simulink model "simulation_4_constant_capacity"  (R2026a)
settings: Solver=VariableStepAuto  StopTime=12000
undefined symbols (not defined in the file): battery_builder_rtmsupport, gcbh
libraries: fl_lib x36, nesl_utility x18, BatteryCurrentManagement x6, Batteries_lib x6, BatteryEstimators x6
(part 2 of 2)

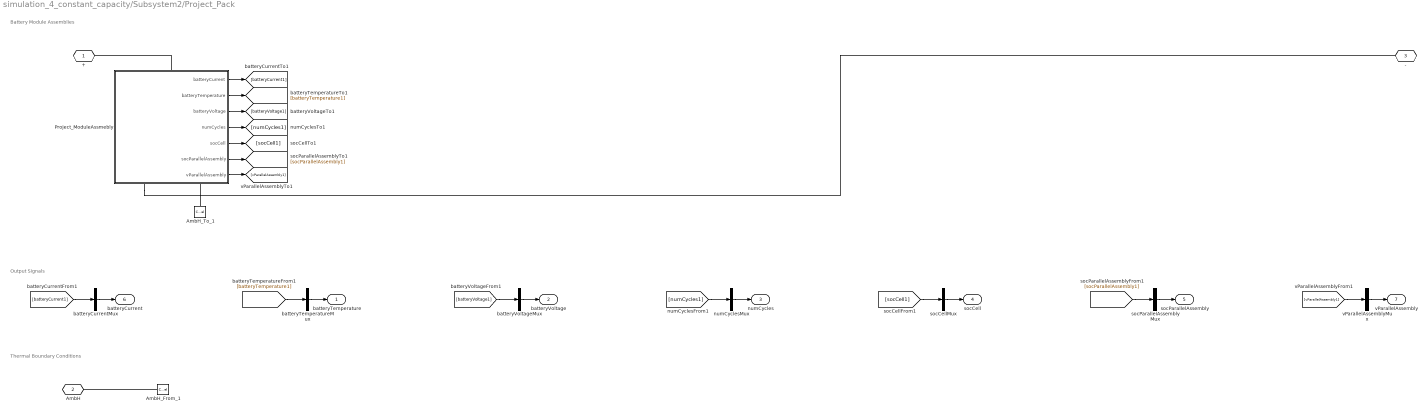
== system simulation_4_constant_capacity/Subsystem2/Project_Pack ==
  note: Thermal Boundary Conditions
  note: Output Signals
  note: Battery Module Assemblies
  AmbH_From_1 : ConnectionLabel  Label=ambH_1
  AmbH_To_1 : ConnectionLabel  Label=ambH_1
  Project_ModuleAssmebly : Subsystem  LoadFcn=battery_builder_rtmsupport('loadfcn',gcbh);
      settings: CopyFcn=battery_builder_rtmsupport('copyfcn',gcbh);  PreCopyFcn=battery_builder_rtmsupport('precopyfcn',gcbh);  PreDeleteFcn=battery_builder_rtmsupport('predeletefcn',gcbh);  PortSchema="{\"entries\":[{\"content\":{\"sides\":[{\"content\":{\"connectorIds\":[\"LConn1\"]},\"type\":\"ConnectorPlacement.EquallySpacedRectSide\",\"uuid\":\"76c6f046-db8e-4015-a922-00ba973faf16\"},{\"content\":{\"connectorIds\":[\"RConn1\",\"RConn2\"],\"side\":\"RIGHT\"},\"type\":\"ConnectorPlacement.EquallySpacedRectSide\",\"uuid\":\"59fdee5c-a6f4-4b44-aa6e-82d2d9418fce\"},{\"content\":{\"side\":\"TOP\"},\"type\":\"ConnectorPlacement.EquallySpacedRectSide\",\"uuid\":\"84b83595-cc1f-46da-a2b0-c16634a6daab\"},{\"content\":{\"connectorIds\":[\"Out1\",\"Out2\",\"Out3\",\"Out4\",\"Out5\",\"Out6\",\"Out7\"],\"side\":\"BOTTOM\"},\"type\":\"ConnectorPlacement.EquallySpacedRectSide\",\"uuid\":\"391f6102-8f79-4306-a331-0bb83eeeb4a2\"}]},\"type\":\"ConnectorPlacement.EquallySpacedConnector\",\"uuid\":\"e6fb231a-8daf-4bfc-bdc1-9175fa7a2dfd\"}],\"packageUris\":[\"http://schema.mathworks.com/mf0/Connector/R2020b\"],\"version\":\"1.0\"}"
      mask Display: image('$imagefile')
  batteryCurrentMux : Mux  Inputs=1
  batteryTemperatureMux : Mux  Inputs=1
  batteryVoltageMux : Mux  Inputs=1
  numCyclesMux : Mux  Inputs=1
  socCellMux : Mux  Inputs=1
  socParallelAssemblyMux : Mux  Inputs=1
  vParallelAssemblyMux : Mux  Inputs=1
  + : PMIOPort  Side=Left
  AmbH : PMIOPort  Port=2  Side=Right  ConnectionType=Connection: foundation.thermal.thermal
  - : PMIOPort  Port=3  Side=Right
  batteryTemperature : Outport
  batteryVoltage : Outport  Port=2
  numCycles : Outport  Port=3
  socCell : Outport  Port=4
  socParallelAssembly : Outport  Port=5
  batteryCurrent : Outport  Port=6
  vParallelAssembly : Outport  Port=7
  wires:
  [vParallelAssembly1] -> vParallelAssemblyMux/1
  vParallelAssemblyMux/1 -> vParallelAssembly/1
  Project_ModuleAssmebly/7(vParallelAssembly) -> [vParallelAssembly1]
  [socParallelAssembly1] -> socParallelAssemblyMux/1
  socParallelAssemblyMux/1 -> socParallelAssembly/1
  Project_ModuleAssmebly/6(socParallelAssembly) -> [socParallelAssembly1]
  [socCell1] -> socCellMux/1
  socCellMux/1 -> socCell/1
  Project_ModuleAssmebly/5(socCell) -> [socCell1]
  [numCycles1] -> numCyclesMux/1
  numCyclesMux/1 -> numCycles/1
  Project_ModuleAssmebly/4(numCycles) -> [numCycles1]
  [batteryVoltage1] -> batteryVoltageMux/1
  batteryVoltageMux/1 -> batteryVoltage/1
  Project_ModuleAssmebly/3(batteryVoltage) -> [batteryVoltage1]
  [batteryTemperature1] -> batteryTemperatureMux/1
  batteryTemperatureMux/1 -> batteryTemperature/1
  Project_ModuleAssmebly/2(batteryTemperature) -> [batteryTemperature1]
  [batteryCurrent1] -> batteryCurrentMux/1
  batteryCurrentMux/1 -> batteryCurrent/1
  Project_ModuleAssmebly/1(batteryCurrent) -> [batteryCurrent1]
  connections:
  AmbH_From_1/LConn1 -- AmbH/RConn1
  AmbH_To_1/LConn1 -- Project_ModuleAssmebly/RConn2
  Project_ModuleAssmebly/RConn1 -- -/RConn1
  Project_ModuleAssmebly/LConn1 -- +/RConn1

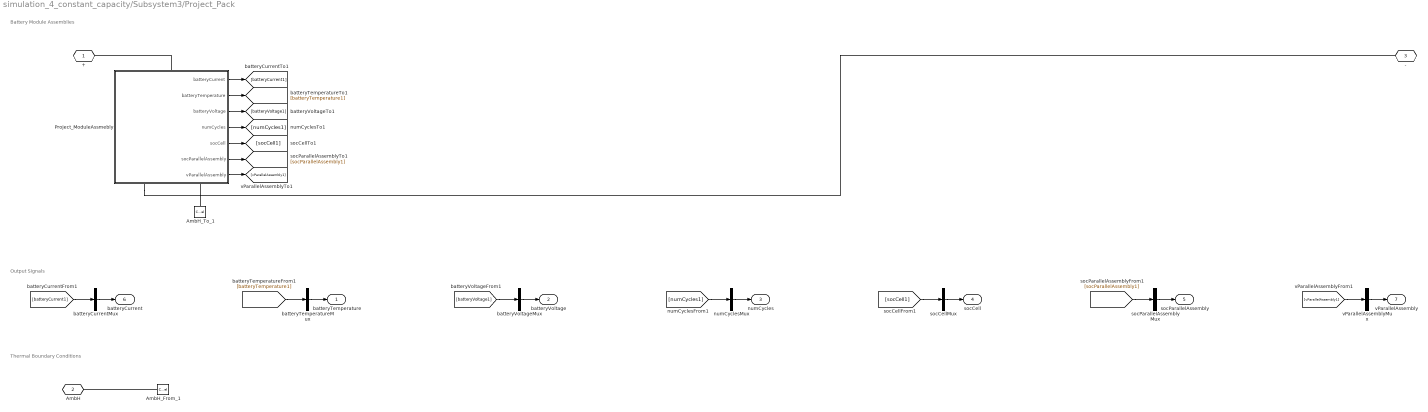
== system simulation_4_constant_capacity/Subsystem3/Project_Pack ==
  note: Thermal Boundary Conditions
  note: Output Signals
  note: Battery Module Assemblies
  AmbH_From_1 : ConnectionLabel  Label=ambH_1
  AmbH_To_1 : ConnectionLabel  Label=ambH_1
  Project_ModuleAssmebly : Subsystem  LoadFcn=battery_builder_rtmsupport('loadfcn',gcbh);
      settings: CopyFcn=battery_builder_rtmsupport('copyfcn',gcbh);  PreCopyFcn=battery_builder_rtmsupport('precopyfcn',gcbh);  PreDeleteFcn=battery_builder_rtmsupport('predeletefcn',gcbh);  PortSchema="{\"entries\":[{\"content\":{\"sides\":[{\"content\":{\"connectorIds\":[\"LConn1\"]},\"type\":\"ConnectorPlacement.EquallySpacedRectSide\",\"uuid\":\"76c6f046-db8e-4015-a922-00ba973faf16\"},{\"content\":{\"connectorIds\":[\"RConn1\",\"RConn2\"],\"side\":\"RIGHT\"},\"type\":\"ConnectorPlacement.EquallySpacedRectSide\",\"uuid\":\"59fdee5c-a6f4-4b44-aa6e-82d2d9418fce\"},{\"content\":{\"side\":\"TOP\"},\"type\":\"ConnectorPlacement.EquallySpacedRectSide\",\"uuid\":\"84b83595-cc1f-46da-a2b0-c16634a6daab\"},{\"content\":{\"connectorIds\":[\"Out1\",\"Out2\",\"Out3\",\"Out4\",\"Out5\",\"Out6\",\"Out7\"],\"side\":\"BOTTOM\"},\"type\":\"ConnectorPlacement.EquallySpacedRectSide\",\"uuid\":\"391f6102-8f79-4306-a331-0bb83eeeb4a2\"}]},\"type\":\"ConnectorPlacement.EquallySpacedConnector\",\"uuid\":\"e6fb231a-8daf-4bfc-bdc1-9175fa7a2dfd\"}],\"packageUris\":[\"http://schema.mathworks.com/mf0/Connector/R2020b\"],\"version\":\"1.0\"}"
      mask Display: image('$imagefile')
  batteryCurrentMux : Mux  Inputs=1
  batteryTemperatureMux : Mux  Inputs=1
  batteryVoltageMux : Mux  Inputs=1
  numCyclesMux : Mux  Inputs=1
  socCellMux : Mux  Inputs=1
  socParallelAssemblyMux : Mux  Inputs=1
  vParallelAssemblyMux : Mux  Inputs=1
  + : PMIOPort  Side=Left
  AmbH : PMIOPort  Port=2  Side=Right  ConnectionType=Connection: foundation.thermal.thermal
  - : PMIOPort  Port=3  Side=Right
  batteryTemperature : Outport
  batteryVoltage : Outport  Port=2
  numCycles : Outport  Port=3
  socCell : Outport  Port=4
  socParallelAssembly : Outport  Port=5
  batteryCurrent : Outport  Port=6
  vParallelAssembly : Outport  Port=7
  wires:
  [vParallelAssembly1] -> vParallelAssemblyMux/1
  vParallelAssemblyMux/1 -> vParallelAssembly/1
  Project_ModuleAssmebly/7(vParallelAssembly) -> [vParallelAssembly1]
  [socParallelAssembly1] -> socParallelAssemblyMux/1
  socParallelAssemblyMux/1 -> socParallelAssembly/1
  Project_ModuleAssmebly/6(socParallelAssembly) -> [socParallelAssembly1]
  [socCell1] -> socCellMux/1
  socCellMux/1 -> socCell/1
  Project_ModuleAssmebly/5(socCell) -> [socCell1]
  [numCycles1] -> numCyclesMux/1
  numCyclesMux/1 -> numCycles/1
  Project_ModuleAssmebly/4(numCycles) -> [numCycles1]
  [batteryVoltage1] -> batteryVoltageMux/1
  batteryVoltageMux/1 -> batteryVoltage/1
  Project_ModuleAssmebly/3(batteryVoltage) -> [batteryVoltage1]
  [batteryTemperature1] -> batteryTemperatureMux/1
  batteryTemperatureMux/1 -> batteryTemperature/1
  Project_ModuleAssmebly/2(batteryTemperature) -> [batteryTemperature1]
  [batteryCurrent1] -> batteryCurrentMux/1
  batteryCurrentMux/1 -> batteryCurrent/1
  Project_ModuleAssmebly/1(batteryCurrent) -> [batteryCurrent1]
  connections:
  AmbH_From_1/LConn1 -- AmbH/RConn1
  AmbH_To_1/LConn1 -- Project_ModuleAssmebly/RConn2
  Project_ModuleAssmebly/RConn1 -- -/RConn1
  Project_ModuleAssmebly/LConn1 -- +/RConn1

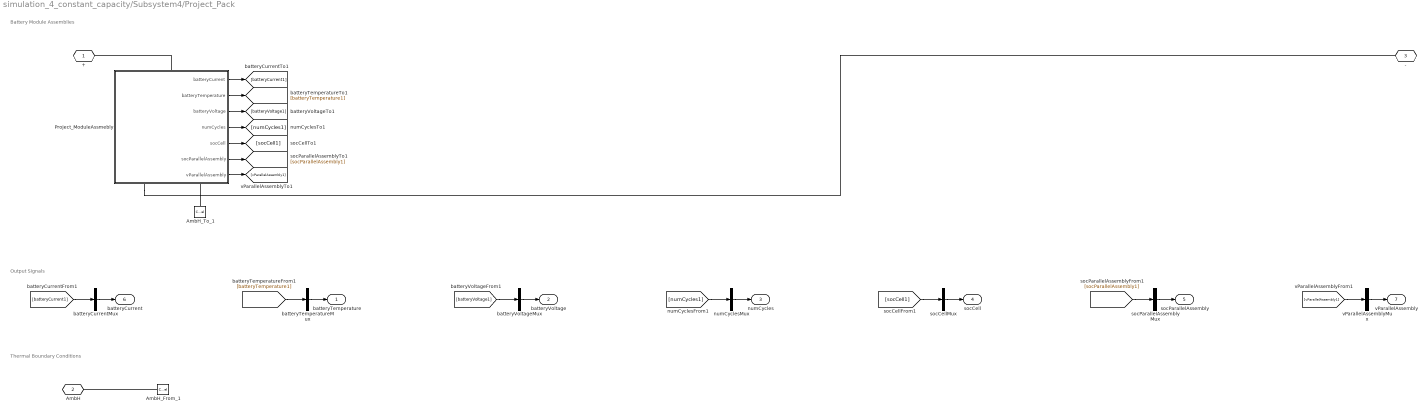
== system simulation_4_constant_capacity/Subsystem4/Project_Pack ==
  note: Thermal Boundary Conditions
  note: Output Signals
  note: Battery Module Assemblies
  AmbH_From_1 : ConnectionLabel  Label=ambH_1
  AmbH_To_1 : ConnectionLabel  Label=ambH_1
  Project_ModuleAssmebly : Subsystem  LoadFcn=battery_builder_rtmsupport('loadfcn',gcbh);
      settings: CopyFcn=battery_builder_rtmsupport('copyfcn',gcbh);  PreCopyFcn=battery_builder_rtmsupport('precopyfcn',gcbh);  PreDeleteFcn=battery_builder_rtmsupport('predeletefcn',gcbh);  PortSchema="{\"entries\":[{\"content\":{\"sides\":[{\"content\":{\"connectorIds\":[\"LConn1\"]},\"type\":\"ConnectorPlacement.EquallySpacedRectSide\",\"uuid\":\"76c6f046-db8e-4015-a922-00ba973faf16\"},{\"content\":{\"connectorIds\":[\"RConn1\",\"RConn2\"],\"side\":\"RIGHT\"},\"type\":\"ConnectorPlacement.EquallySpacedRectSide\",\"uuid\":\"59fdee5c-a6f4-4b44-aa6e-82d2d9418fce\"},{\"content\":{\"side\":\"TOP\"},\"type\":\"ConnectorPlacement.EquallySpacedRectSide\",\"uuid\":\"84b83595-cc1f-46da-a2b0-c16634a6daab\"},{\"content\":{\"connectorIds\":[\"Out1\",\"Out2\",\"Out3\",\"Out4\",\"Out5\",\"Out6\",\"Out7\"],\"side\":\"BOTTOM\"},\"type\":\"ConnectorPlacement.EquallySpacedRectSide\",\"uuid\":\"391f6102-8f79-4306-a331-0bb83eeeb4a2\"}]},\"type\":\"ConnectorPlacement.EquallySpacedConnector\",\"uuid\":\"e6fb231a-8daf-4bfc-bdc1-9175fa7a2dfd\"}],\"packageUris\":[\"http://schema.mathworks.com/mf0/Connector/R2020b\"],\"version\":\"1.0\"}"
      mask Display: image('$imagefile')
  batteryCurrentMux : Mux  Inputs=1
  batteryTemperatureMux : Mux  Inputs=1
  batteryVoltageMux : Mux  Inputs=1
  numCyclesMux : Mux  Inputs=1
  socCellMux : Mux  Inputs=1
  socParallelAssemblyMux : Mux  Inputs=1
  vParallelAssemblyMux : Mux  Inputs=1
  + : PMIOPort  Side=Left
  AmbH : PMIOPort  Port=2  Side=Right  ConnectionType=Connection: foundation.thermal.thermal
  - : PMIOPort  Port=3  Side=Right
  batteryTemperature : Outport
  batteryVoltage : Outport  Port=2
  numCycles : Outport  Port=3
  socCell : Outport  Port=4
  socParallelAssembly : Outport  Port=5
  batteryCurrent : Outport  Port=6
  vParallelAssembly : Outport  Port=7
  wires:
  [vParallelAssembly1] -> vParallelAssemblyMux/1
  vParallelAssemblyMux/1 -> vParallelAssembly/1
  Project_ModuleAssmebly/7(vParallelAssembly) -> [vParallelAssembly1]
  [socParallelAssembly1] -> socParallelAssemblyMux/1
  socParallelAssemblyMux/1 -> socParallelAssembly/1
  Project_ModuleAssmebly/6(socParallelAssembly) -> [socParallelAssembly1]
  [socCell1] -> socCellMux/1
  socCellMux/1 -> socCell/1
  Project_ModuleAssmebly/5(socCell) -> [socCell1]
  [numCycles1] -> numCyclesMux/1
  numCyclesMux/1 -> numCycles/1
  Project_ModuleAssmebly/4(numCycles) -> [numCycles1]
  [batteryVoltage1] -> batteryVoltageMux/1
  batteryVoltageMux/1 -> batteryVoltage/1
  Project_ModuleAssmebly/3(batteryVoltage) -> [batteryVoltage1]
  [batteryTemperature1] -> batteryTemperatureMux/1
  batteryTemperatureMux/1 -> batteryTemperature/1
  Project_ModuleAssmebly/2(batteryTemperature) -> [batteryTemperature1]
  [batteryCurrent1] -> batteryCurrentMux/1
  batteryCurrentMux/1 -> batteryCurrent/1
  Project_ModuleAssmebly/1(batteryCurrent) -> [batteryCurrent1]
  connections:
  AmbH_From_1/LConn1 -- AmbH/RConn1
  AmbH_To_1/LConn1 -- Project_ModuleAssmebly/RConn2
  Project_ModuleAssmebly/RConn1 -- -/RConn1
  Project_ModuleAssmebly/LConn1 -- +/RConn1

== system simulation_4_constant_capacity/Subsystem5/Project_Pack ==
  note: Thermal Boundary Conditions
  note: Output Signals
  note: Battery Module Assemblies
  AmbH_From_1 : ConnectionLabel  Label=ambH_1
  AmbH_To_1 : ConnectionLabel  Label=ambH_1
  Project_ModuleAssmebly : Subsystem  LoadFcn=battery_builder_rtmsupport('loadfcn',gcbh);
      settings: CopyFcn=battery_builder_rtmsupport('copyfcn',gcbh);  PreCopyFcn=battery_builder_rtmsupport('precopyfcn',gcbh);  PreDeleteFcn=battery_builder_rtmsupport('predeletefcn',gcbh);  PortSchema="{\"entries\":[{\"content\":{\"sides\":[{\"content\":{\"connectorIds\":[\"LConn1\"]},\"type\":\"ConnectorPlacement.EquallySpacedRectSide\",\"uuid\":\"76c6f046-db8e-4015-a922-00ba973faf16\"},{\"content\":{\"connectorIds\":[\"RConn1\",\"RConn2\"],\"side\":\"RIGHT\"},\"type\":\"ConnectorPlacement.EquallySpacedRectSide\",\"uuid\":\"59fdee5c-a6f4-4b44-aa6e-82d2d9418fce\"},{\"content\":{\"side\":\"TOP\"},\"type\":\"ConnectorPlacement.EquallySpacedRectSide\",\"uuid\":\"84b83595-cc1f-46da-a2b0-c16634a6daab\"},{\"content\":{\"connectorIds\":[\"Out1\",\"Out2\",\"Out3\",\"Out4\",\"Out5\",\"Out6\",\"Out7\"],\"side\":\"BOTTOM\"},\"type\":\"ConnectorPlacement.EquallySpacedRectSide\",\"uuid\":\"391f6102-8f79-4306-a331-0bb83eeeb4a2\"}]},\"type\":\"ConnectorPlacement.EquallySpacedConnector\",\"uuid\":\"e6fb231a-8daf-4bfc-bdc1-9175fa7a2dfd\"}],\"packageUris\":[\"http://schema.mathworks.com/mf0/Connector/R2020b\"],\"version\":\"1.0\"}"
      mask Display: image('$imagefile')
  batteryCurrentMux : Mux  Inputs=1
  batteryTemperatureMux : Mux  Inputs=1
  batteryVoltageMux : Mux  Inputs=1
  numCyclesMux : Mux  Inputs=1
  socCellMux : Mux  Inputs=1
  socParallelAssemblyMux : Mux  Inputs=1
  vParallelAssemblyMux : Mux  Inputs=1
  + : PMIOPort  Side=Left
  AmbH : PMIOPort  Port=2  Side=Right  ConnectionType=Connection: foundation.thermal.thermal
  - : PMIOPort  Port=3  Side=Right
  batteryTemperature : Outport
  batteryVoltage : Outport  Port=2
  numCycles : Outport  Port=3
  socCell : Outport  Port=4
  socParallelAssembly : Outport  Port=5
  batteryCurrent : Outport  Port=6
  vParallelAssembly : Outport  Port=7
  wires:
  [vParallelAssembly1] -> vParallelAssemblyMux/1
  vParallelAssemblyMux/1 -> vParallelAssembly/1
  Project_ModuleAssmebly/7(vParallelAssembly) -> [vParallelAssembly1]
  [socParallelAssembly1] -> socParallelAssemblyMux/1
  socParallelAssemblyMux/1 -> socParallelAssembly/1
  Project_ModuleAssmebly/6(socParallelAssembly) -> [socParallelAssembly1]
  [socCell1] -> socCellMux/1
  socCellMux/1 -> socCell/1
  Project_ModuleAssmebly/5(socCell) -> [socCell1]
  [numCycles1] -> numCyclesMux/1
  numCyclesMux/1 -> numCycles/1
  Project_ModuleAssmebly/4(numCycles) -> [numCycles1]
  [batteryVoltage1] -> batteryVoltageMux/1
  batteryVoltageMux/1 -> batteryVoltage/1
  Project_ModuleAssmebly/3(batteryVoltage) -> [batteryVoltage1]
  [batteryTemperature1] -> batteryTemperatureMux/1
  batteryTemperatureMux/1 -> batteryTemperature/1
  Project_ModuleAssmebly/2(batteryTemperature) -> [batteryTemperature1]
  [batteryCurrent1] -> batteryCurrentMux/1
  batteryCurrentMux/1 -> batteryCurrent/1
  Project_ModuleAssmebly/1(batteryCurrent) -> [batteryCurrent1]
  connections:
  AmbH_From_1/LConn1 -- AmbH/RConn1
  AmbH_To_1/LConn1 -- Project_ModuleAssmebly/RConn2
  Project_ModuleAssmebly/RConn1 -- -/RConn1
  Project_ModuleAssmebly/LConn1 -- +/RConn1

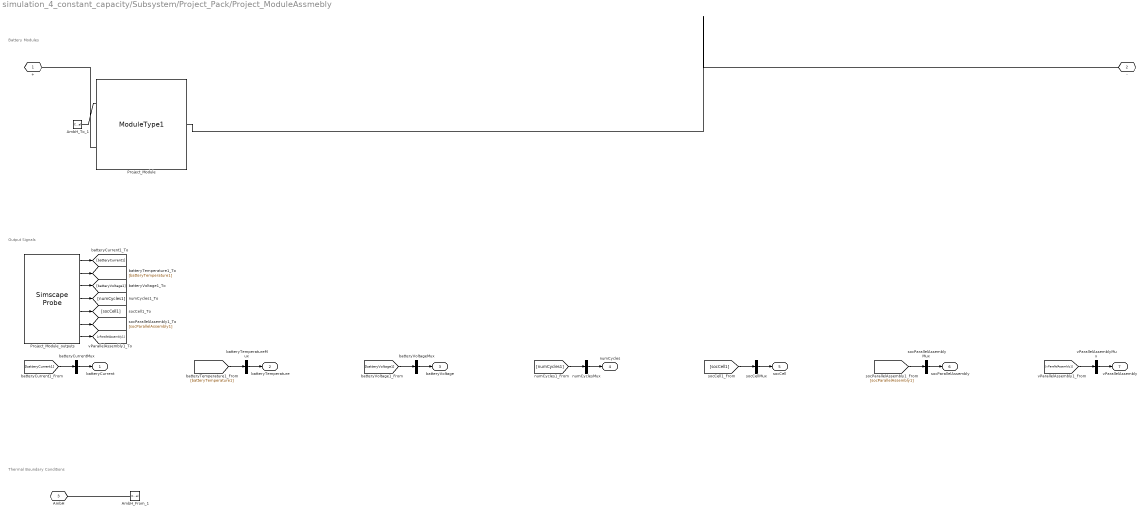
== system simulation_4_constant_capacity/Subsystem/Project_Pack/Project_ModuleAssmebly ==
  note: Battery Modules
  note: Output Signals
  note: Thermal Boundary Conditions
  AmbH_From_1 : ConnectionLabel  Label=ambH_1
  AmbH_To_1 : ConnectionLabel  Label=ambH_1
  Project_Module : Batteries_lib/Modules/ModuleType1  BatteryCapacityCell=2.6 A*hr  ExtrapolationMethodCell=simscape.enum.extrapolation.nearest  SOCBreakpointsCell=[0 0.1 0.2 0.3 0.4 0.5 0.6 0.7 0.8 0.9 1]  TemperatureBreakpointsCell=[253.15 263.15 273.15 296.15 318.15] K  OpenCircuitVoltageThermalCell=|  VoltageRangeCell=[0, inf] V  ResistanceSOCBreakpointsCell=[0, .1, .25, .5, .75, .9, 1]  ResistanceTemperatureBreakpointsCell=[278, 293, 313] K  R0ThermalCell=[.0117, .0085, .009; .011, .0085, .009; .0114, .0087, .0092; .0107, .0082, .0088; .0107, .0083, .0091; .0113, .0085, .0089; .0116, .0085, .0089] Ohm  BatteryThermalMassCell=1840 J/K  AmbientResistance=25 K/W  socCell_specify=off  socCell_priority=High  socCell=0  socCell_nominal_specify=off  socCell_nominal_value=1  socCell_nominal_unit=1  batteryVoltage_specify=off  batteryVoltage_priority=None  batteryVoltage=0 V  batteryVoltage_nominal_specify=off  batteryVoltage_nominal_value=1  batteryVoltage_nominal_unit=V  batteryCurrent_specify=off  batteryCurrent_priority=None  batteryCurrent=0 A  batteryCurrent_nominal_specify=off  batteryCurrent_nominal_value=1  batteryCurrent_nominal_unit=A  numCycles_specify=off  numCycles_priority=High  numCycles=0  numCycles_nominal_specify=off  numCycles_nominal_value=1  numCycles_nominal_unit=1  batteryTemperature_specify=on  batteryTemperature_priority=High  batteryTemperature=258 K  batteryTemperature_nominal_specify=off  batteryTemperature_nominal_value=1  batteryTemperature_nominal_unit=K  vParallelAssembly_specify=off  vParallelAssembly_priority=None  vParallelAssembly=repmat(0, 10, 1) V  vParallelAssembly_nominal_specify=off  vParallelAssembly_nominal_value=1  vParallelAssembly_nominal_unit=V  socParallelAssembly_specify=off  socParallelAssembly_priority=None  socParallelAssembly=repmat(1, 10, 1)  socParallelAssembly_nominal_specify=off  socParallelAssembly_nominal_value=1  socParallelAssembly_nominal_unit=1
      | [3.00 3.00 3.00 3.00 3.00;
      |  3.07 3.23 3.40 3.65 3.70;
      |  3.09 3.31 3.49 3.67 3.71;
      |  3.10 3.38 3.54 3.70 3.73;
      |  3.11 3.44 3.59 3.72 3.75;
      |  3.13 3.50 3.65 3.75 3.78;
      |  3.15 3.55 3.70 3.80 3.83;
      |  3.19 3.61 3.76 3.87 3.90;
      |  3.24 3.69 3.82 3.95 3.98;
      |  3.34 3.78 3.90 4.02 4.03;
      |  3.59 3.97 4.10 4.16 4.16] V
  Project_Module_outputs : SimscapeProbe  BoundBlock=482  Variables="{\"batteryCurrent\":{\"Probing\":\"ON\"},\"batteryTemperature\":{\"Probing\":\"ON\"},\"batteryVoltage\":{\"Probing\":\"ON\"},\"numCycles\":{\"Probing\":\"ON\"},\"socCell\":{\"Probing\":\"ON\"},\"socParallelAssembly\":{\"Probing\":\"ON\"},\"vParallelAssembly\":{\"Probing\":\"ON\"}}"
  batteryCurrentMux : Mux  Inputs=1
  batteryTemperatureMux : Mux  Inputs=1
  batteryVoltageMux : Mux  Inputs=1
  numCyclesMux : Mux  Inputs=1
  socCellMux : Mux  Inputs=1
  socParallelAssemblyMux : Mux  Inputs=1
  vParallelAssemblyMux : Mux  Inputs=1
  + : PMIOPort  Side=Left
  - : PMIOPort  Port=2  Side=Right
  AmbH : PMIOPort  Port=3  Side=Right  ConnectionType=Connection: foundation.thermal.thermal
  batteryCurrent : Outport
  batteryTemperature : Outport  Port=2
  batteryVoltage : Outport  Port=3
  numCycles : Outport  Port=4
  socCell : Outport  Port=5
  socParallelAssembly : Outport  Port=6
  vParallelAssembly : Outport  Port=7
  wires:
  Project_Module_outputs/1 -> [batteryCurrent1]
  batteryCurrentMux/1 -> batteryCurrent/1
  [batteryCurrent1] -> batteryCurrentMux/1
  Project_Module_outputs/2 -> [batteryTemperature1]
  batteryTemperatureMux/1 -> batteryTemperature/1
  [batteryTemperature1] -> batteryTemperatureMux/1
  Project_Module_outputs/3 -> [batteryVoltage1]
  batteryVoltageMux/1 -> batteryVoltage/1
  [batteryVoltage1] -> batteryVoltageMux/1
  Project_Module_outputs/4 -> [numCycles1]
  numCyclesMux/1 -> numCycles/1
  [numCycles1] -> numCyclesMux/1
  Project_Module_outputs/5 -> [socCell1]
  socCellMux/1 -> socCell/1
  [socCell1] -> socCellMux/1
  Project_Module_outputs/6 -> [socParallelAssembly1]
  socParallelAssemblyMux/1 -> socParallelAssembly/1
  [socParallelAssembly1] -> socParallelAssemblyMux/1
  Project_Module_outputs/7 -> [vParallelAssembly1]
  vParallelAssemblyMux/1 -> vParallelAssembly/1
  [vParallelAssembly1] -> vParallelAssemblyMux/1
  connections:
  Project_Module/LConn2 -- +/RConn1
  Project_Module/RConn1 -- -/RConn1
  AmbH_To_1/LConn1 -- Project_Module/LConn1
  AmbH_From_1/LConn1 -- AmbH/RConn1

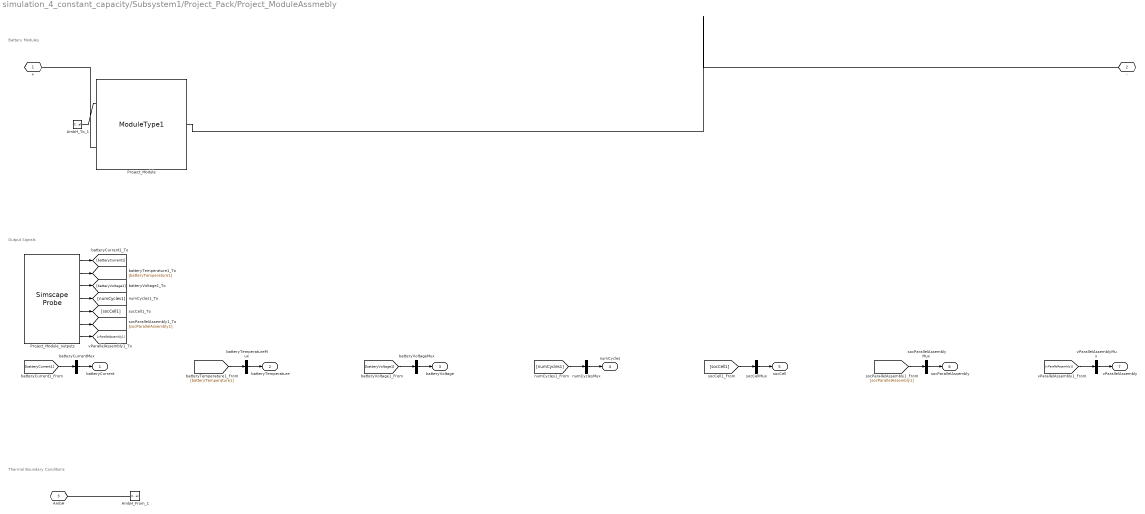
== system simulation_4_constant_capacity/Subsystem1/Project_Pack/Project_ModuleAssmebly ==
  note: Battery Modules
  note: Output Signals
  note: Thermal Boundary Conditions
  AmbH_From_1 : ConnectionLabel  Label=ambH_1
  AmbH_To_1 : ConnectionLabel  Label=ambH_1
  Project_Module : Batteries_lib/Modules/ModuleType1  BatteryCapacityCell=2.6 A*hr  ExtrapolationMethodCell=simscape.enum.extrapolation.nearest  SOCBreakpointsCell=[0 0.1 0.2 0.3 0.4 0.5 0.6 0.7 0.8 0.9 1]  TemperatureBreakpointsCell=[253.15 263.15 273.15 296.15 318.15] K  OpenCircuitVoltageThermalCell=|  VoltageRangeCell=[0, inf] V  ResistanceSOCBreakpointsCell=[0, .1, .25, .5, .75, .9, 1]  ResistanceTemperatureBreakpointsCell=[278, 293, 313] K  R0ThermalCell=[.0117, .0085, .009; .011, .0085, .009; .0114, .0087, .0092; .0107, .0082, .0088; .0107, .0083, .0091; .0113, .0085, .0089; .0116, .0085, .0089] Ohm  BatteryThermalMassCell=1840 J/K  AmbientResistance=25 K/W  socCell_specify=off  socCell_priority=High  socCell=0  socCell_nominal_specify=off  socCell_nominal_value=1  socCell_nominal_unit=1  batteryVoltage_specify=off  batteryVoltage_priority=None  batteryVoltage=0 V  batteryVoltage_nominal_specify=off  batteryVoltage_nominal_value=1  batteryVoltage_nominal_unit=V  batteryCurrent_specify=off  batteryCurrent_priority=None  batteryCurrent=0 A  batteryCurrent_nominal_specify=off  batteryCurrent_nominal_value=1  batteryCurrent_nominal_unit=A  numCycles_specify=off  numCycles_priority=High  numCycles=0  numCycles_nominal_specify=off  numCycles_nominal_value=1  numCycles_nominal_unit=1  batteryTemperature_specify=on  batteryTemperature_priority=High  batteryTemperature=248 K  batteryTemperature_nominal_specify=off  batteryTemperature_nominal_value=1  batteryTemperature_nominal_unit=K  vParallelAssembly_specify=off  vParallelAssembly_priority=None  vParallelAssembly=repmat(0, 10, 1) V  vParallelAssembly_nominal_specify=off  vParallelAssembly_nominal_value=1  vParallelAssembly_nominal_unit=V  socParallelAssembly_specify=off  socParallelAssembly_priority=None  socParallelAssembly=repmat(1, 10, 1)  socParallelAssembly_nominal_specify=off  socParallelAssembly_nominal_value=1  socParallelAssembly_nominal_unit=1
      | [3.00 3.00 3.00 3.00 3.00;
      |  3.07 3.23 3.40 3.65 3.70;
      |  3.09 3.31 3.49 3.67 3.71;
      |  3.10 3.38 3.54 3.70 3.73;
      |  3.11 3.44 3.59 3.72 3.75;
      |  3.13 3.50 3.65 3.75 3.78;
      |  3.15 3.55 3.70 3.80 3.83;
      |  3.19 3.61 3.76 3.87 3.90;
      |  3.24 3.69 3.82 3.95 3.98;
      |  3.34 3.78 3.90 4.02 4.03;
      |  3.59 3.97 4.10 4.16 4.16] V
  Project_Module_outputs : SimscapeProbe  BoundBlock=909  Variables="{\"batteryCurrent\":{\"Probing\":\"ON\"},\"batteryTemperature\":{\"Probing\":\"ON\"},\"batteryVoltage\":{\"Probing\":\"ON\"},\"numCycles\":{\"Probing\":\"ON\"},\"socCell\":{\"Probing\":\"ON\"},\"socParallelAssembly\":{\"Probing\":\"ON\"},\"vParallelAssembly\":{\"Probing\":\"ON\"}}"
  batteryCurrentMux : Mux  Inputs=1
  batteryTemperatureMux : Mux  Inputs=1
  batteryVoltageMux : Mux  Inputs=1
  numCyclesMux : Mux  Inputs=1
  socCellMux : Mux  Inputs=1
  socParallelAssemblyMux : Mux  Inputs=1
  vParallelAssemblyMux : Mux  Inputs=1
  + : PMIOPort  Side=Left
  - : PMIOPort  Port=2  Side=Right
  AmbH : PMIOPort  Port=3  Side=Right  ConnectionType=Connection: foundation.thermal.thermal
  batteryCurrent : Outport
  batteryTemperature : Outport  Port=2
  batteryVoltage : Outport  Port=3
  numCycles : Outport  Port=4
  socCell : Outport  Port=5
  socParallelAssembly : Outport  Port=6
  vParallelAssembly : Outport  Port=7
  wires:
  Project_Module_outputs/1 -> [batteryCurrent1]
  batteryCurrentMux/1 -> batteryCurrent/1
  [batteryCurrent1] -> batteryCurrentMux/1
  Project_Module_outputs/2 -> [batteryTemperature1]
  batteryTemperatureMux/1 -> batteryTemperature/1
  [batteryTemperature1] -> batteryTemperatureMux/1
  Project_Module_outputs/3 -> [batteryVoltage1]
  batteryVoltageMux/1 -> batteryVoltage/1
  [batteryVoltage1] -> batteryVoltageMux/1
  Project_Module_outputs/4 -> [numCycles1]
  numCyclesMux/1 -> numCycles/1
  [numCycles1] -> numCyclesMux/1
  Project_Module_outputs/5 -> [socCell1]
  socCellMux/1 -> socCell/1
  [socCell1] -> socCellMux/1
  Project_Module_outputs/6 -> [socParallelAssembly1]
  socParallelAssemblyMux/1 -> socParallelAssembly/1
  [socParallelAssembly1] -> socParallelAssemblyMux/1
  Project_Module_outputs/7 -> [vParallelAssembly1]
  vParallelAssemblyMux/1 -> vParallelAssembly/1
  [vParallelAssembly1] -> vParallelAssemblyMux/1
  connections:
  Project_Module/LConn2 -- +/RConn1
  Project_Module/RConn1 -- -/RConn1
  AmbH_To_1/LConn1 -- Project_Module/LConn1
  AmbH_From_1/LConn1 -- AmbH/RConn1

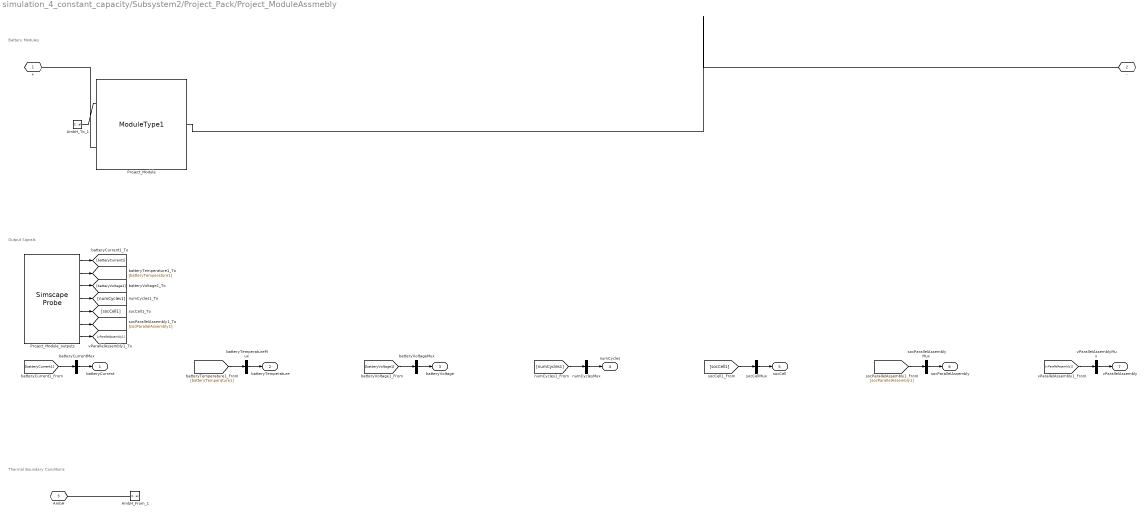
== system simulation_4_constant_capacity/Subsystem2/Project_Pack/Project_ModuleAssmebly ==
  note: Battery Modules
  note: Output Signals
  note: Thermal Boundary Conditions
  AmbH_From_1 : ConnectionLabel  Label=ambH_1
  AmbH_To_1 : ConnectionLabel  Label=ambH_1
  Project_Module : Batteries_lib/Modules/ModuleType1  BatteryCapacityCell=2.6 A*hr  ExtrapolationMethodCell=simscape.enum.extrapolation.nearest  SOCBreakpointsCell=[0 0.1 0.2 0.3 0.4 0.5 0.6 0.7 0.8 0.9 1]  TemperatureBreakpointsCell=[253.15 263.15 273.15 296.15 318.15] K  OpenCircuitVoltageThermalCell=|  VoltageRangeCell=[0, inf] V  ResistanceSOCBreakpointsCell=[0, .1, .25, .5, .75, .9, 1]  ResistanceTemperatureBreakpointsCell=[278, 293, 313] K  R0ThermalCell=[.0117, .0085, .009; .011, .0085, .009; .0114, .0087, .0092; .0107, .0082, .0088; .0107, .0083, .0091; .0113, .0085, .0089; .0116, .0085, .0089] Ohm  BatteryThermalMassCell=1840 J/K  AmbientResistance=25 K/W  socCell_specify=off  socCell_priority=High  socCell=0  socCell_nominal_specify=off  socCell_nominal_value=1  socCell_nominal_unit=1  batteryVoltage_specify=off  batteryVoltage_priority=None  batteryVoltage=0 V  batteryVoltage_nominal_specify=off  batteryVoltage_nominal_value=1  batteryVoltage_nominal_unit=V  batteryCurrent_specify=off  batteryCurrent_priority=None  batteryCurrent=0 A  batteryCurrent_nominal_specify=off  batteryCurrent_nominal_value=1  batteryCurrent_nominal_unit=A  numCycles_specify=off  numCycles_priority=High  numCycles=0  numCycles_nominal_specify=off  numCycles_nominal_value=1  numCycles_nominal_unit=1  batteryTemperature_specify=on  batteryTemperature_priority=High  batteryTemperature=268 K  batteryTemperature_nominal_specify=off  batteryTemperature_nominal_value=1  batteryTemperature_nominal_unit=K  vParallelAssembly_specify=off  vParallelAssembly_priority=None  vParallelAssembly=repmat(0, 10, 1) V  vParallelAssembly_nominal_specify=off  vParallelAssembly_nominal_value=1  vParallelAssembly_nominal_unit=V  socParallelAssembly_specify=off  socParallelAssembly_priority=None  socParallelAssembly=repmat(1, 10, 1)  socParallelAssembly_nominal_specify=off  socParallelAssembly_nominal_value=1  socParallelAssembly_nominal_unit=1
      | [3.00 3.00 3.00 3.00 3.00;
      |  3.07 3.23 3.40 3.65 3.70;
      |  3.09 3.31 3.49 3.67 3.71;
      |  3.10 3.38 3.54 3.70 3.73;
      |  3.11 3.44 3.59 3.72 3.75;
      |  3.13 3.50 3.65 3.75 3.78;
      |  3.15 3.55 3.70 3.80 3.83;
      |  3.19 3.61 3.76 3.87 3.90;
      |  3.24 3.69 3.82 3.95 3.98;
      |  3.34 3.78 3.90 4.02 4.03;
      |  3.59 3.97 4.10 4.16 4.16] V
  Project_Module_outputs : SimscapeProbe  BoundBlock=1014  Variables="{\"batteryCurrent\":{\"Probing\":\"ON\"},\"batteryTemperature\":{\"Probing\":\"ON\"},\"batteryVoltage\":{\"Probing\":\"ON\"},\"numCycles\":{\"Probing\":\"ON\"},\"socCell\":{\"Probing\":\"ON\"},\"socParallelAssembly\":{\"Probing\":\"ON\"},\"vParallelAssembly\":{\"Probing\":\"ON\"}}"
  batteryCurrentMux : Mux  Inputs=1
  batteryTemperatureMux : Mux  Inputs=1
  batteryVoltageMux : Mux  Inputs=1
  numCyclesMux : Mux  Inputs=1
  socCellMux : Mux  Inputs=1
  socParallelAssemblyMux : Mux  Inputs=1
  vParallelAssemblyMux : Mux  Inputs=1
  + : PMIOPort  Side=Left
  - : PMIOPort  Port=2  Side=Right
  AmbH : PMIOPort  Port=3  Side=Right  ConnectionType=Connection: foundation.thermal.thermal
  batteryCurrent : Outport
  batteryTemperature : Outport  Port=2
  batteryVoltage : Outport  Port=3
  numCycles : Outport  Port=4
  socCell : Outport  Port=5
  socParallelAssembly : Outport  Port=6
  vParallelAssembly : Outport  Port=7
  wires:
  Project_Module_outputs/1 -> [batteryCurrent1]
  batteryCurrentMux/1 -> batteryCurrent/1
  [batteryCurrent1] -> batteryCurrentMux/1
  Project_Module_outputs/2 -> [batteryTemperature1]
  batteryTemperatureMux/1 -> batteryTemperature/1
  [batteryTemperature1] -> batteryTemperatureMux/1
  Project_Module_outputs/3 -> [batteryVoltage1]
  batteryVoltageMux/1 -> batteryVoltage/1
  [batteryVoltage1] -> batteryVoltageMux/1
  Project_Module_outputs/4 -> [numCycles1]
  numCyclesMux/1 -> numCycles/1
  [numCycles1] -> numCyclesMux/1
  Project_Module_outputs/5 -> [socCell1]
  socCellMux/1 -> socCell/1
  [socCell1] -> socCellMux/1
  Project_Module_outputs/6 -> [socParallelAssembly1]
  socParallelAssemblyMux/1 -> socParallelAssembly/1
  [socParallelAssembly1] -> socParallelAssemblyMux/1
  Project_Module_outputs/7 -> [vParallelAssembly1]
  vParallelAssemblyMux/1 -> vParallelAssembly/1
  [vParallelAssembly1] -> vParallelAssemblyMux/1
  connections:
  Project_Module/LConn2 -- +/RConn1
  Project_Module/RConn1 -- -/RConn1
  AmbH_To_1/LConn1 -- Project_Module/LConn1
  AmbH_From_1/LConn1 -- AmbH/RConn1

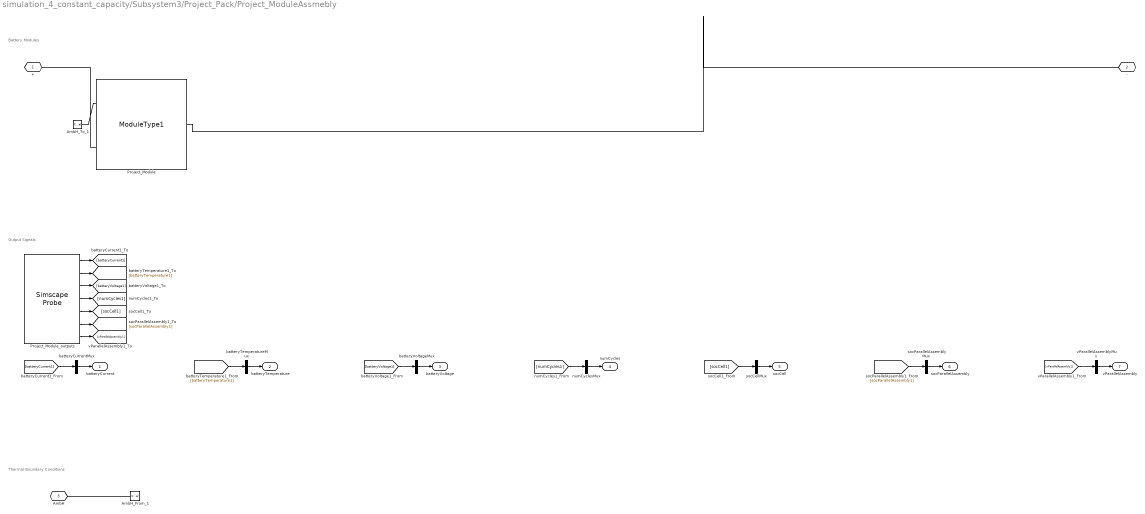
== system simulation_4_constant_capacity/Subsystem3/Project_Pack/Project_ModuleAssmebly ==
  note: Battery Modules
  note: Output Signals
  note: Thermal Boundary Conditions
  AmbH_From_1 : ConnectionLabel  Label=ambH_1
  AmbH_To_1 : ConnectionLabel  Label=ambH_1
  Project_Module : Batteries_lib/Modules/ModuleType1  BatteryCapacityCell=2.6 A*hr  ExtrapolationMethodCell=simscape.enum.extrapolation.nearest  SOCBreakpointsCell=[0 0.1 0.2 0.3 0.4 0.5 0.6 0.7 0.8 0.9 1]  TemperatureBreakpointsCell=[253.15 263.15 273.15 296.15 318.15] K  OpenCircuitVoltageThermalCell=|  VoltageRangeCell=[0, inf] V  ResistanceSOCBreakpointsCell=[0, .1, .25, .5, .75, .9, 1]  ResistanceTemperatureBreakpointsCell=[278, 293, 313] K  R0ThermalCell=[.0117, .0085, .009; .011, .0085, .009; .0114, .0087, .0092; .0107, .0082, .0088; .0107, .0083, .0091; .0113, .0085, .0089; .0116, .0085, .0089] Ohm  BatteryThermalMassCell=1840 J/K  AmbientResistance=25 K/W  socCell_specify=off  socCell_priority=High  socCell=0  socCell_nominal_specify=off  socCell_nominal_value=1  socCell_nominal_unit=1  batteryVoltage_specify=off  batteryVoltage_priority=None  batteryVoltage=0 V  batteryVoltage_nominal_specify=off  batteryVoltage_nominal_value=1  batteryVoltage_nominal_unit=V  batteryCurrent_specify=off  batteryCurrent_priority=None  batteryCurrent=0 A  batteryCurrent_nominal_specify=off  batteryCurrent_nominal_value=1  batteryCurrent_nominal_unit=A  numCycles_specify=off  numCycles_priority=High  numCycles=0  numCycles_nominal_specify=off  numCycles_nominal_value=1  numCycles_nominal_unit=1  batteryTemperature_specify=on  batteryTemperature_priority=High  batteryTemperature=303 K  batteryTemperature_nominal_specify=off  batteryTemperature_nominal_value=1  batteryTemperature_nominal_unit=K  vParallelAssembly_specify=off  vParallelAssembly_priority=None  vParallelAssembly=repmat(0, 10, 1) V  vParallelAssembly_nominal_specify=off  vParallelAssembly_nominal_value=1  vParallelAssembly_nominal_unit=V  socParallelAssembly_specify=off  socParallelAssembly_priority=None  socParallelAssembly=repmat(1, 10, 1)  socParallelAssembly_nominal_specify=off  socParallelAssembly_nominal_value=1  socParallelAssembly_nominal_unit=1
      | [3.00 3.00 3.00 3.00 3.00;
      |  3.07 3.23 3.40 3.65 3.70;
      |  3.09 3.31 3.49 3.67 3.71;
      |  3.10 3.38 3.54 3.70 3.73;
      |  3.11 3.44 3.59 3.72 3.75;
      |  3.13 3.50 3.65 3.75 3.78;
      |  3.15 3.55 3.70 3.80 3.83;
      |  3.19 3.61 3.76 3.87 3.90;
      |  3.24 3.69 3.82 3.95 3.98;
      |  3.34 3.78 3.90 4.02 4.03;
      |  3.59 3.97 4.10 4.16 4.16] V
  Project_Module_outputs : SimscapeProbe  BoundBlock=1119  Variables="{\"batteryCurrent\":{\"Probing\":\"ON\"},\"batteryTemperature\":{\"Probing\":\"ON\"},\"batteryVoltage\":{\"Probing\":\"ON\"},\"numCycles\":{\"Probing\":\"ON\"},\"socCell\":{\"Probing\":\"ON\"},\"socParallelAssembly\":{\"Probing\":\"ON\"},\"vParallelAssembly\":{\"Probing\":\"ON\"}}"
  batteryCurrentMux : Mux  Inputs=1
  batteryTemperatureMux : Mux  Inputs=1
  batteryVoltageMux : Mux  Inputs=1
  numCyclesMux : Mux  Inputs=1
  socCellMux : Mux  Inputs=1
  socParallelAssemblyMux : Mux  Inputs=1
  vParallelAssemblyMux : Mux  Inputs=1
  + : PMIOPort  Side=Left
  - : PMIOPort  Port=2  Side=Right
  AmbH : PMIOPort  Port=3  Side=Right  ConnectionType=Connection: foundation.thermal.thermal
  batteryCurrent : Outport
  batteryTemperature : Outport  Port=2
  batteryVoltage : Outport  Port=3
  numCycles : Outport  Port=4
  socCell : Outport  Port=5
  socParallelAssembly : Outport  Port=6
  vParallelAssembly : Outport  Port=7
  wires:
  Project_Module_outputs/1 -> [batteryCurrent1]
  batteryCurrentMux/1 -> batteryCurrent/1
  [batteryCurrent1] -> batteryCurrentMux/1
  Project_Module_outputs/2 -> [batteryTemperature1]
  batteryTemperatureMux/1 -> batteryTemperature/1
  [batteryTemperature1] -> batteryTemperatureMux/1
  Project_Module_outputs/3 -> [batteryVoltage1]
  batteryVoltageMux/1 -> batteryVoltage/1
  [batteryVoltage1] -> batteryVoltageMux/1
  Project_Module_outputs/4 -> [numCycles1]
  numCyclesMux/1 -> numCycles/1
  [numCycles1] -> numCyclesMux/1
  Project_Module_outputs/5 -> [socCell1]
  socCellMux/1 -> socCell/1
  [socCell1] -> socCellMux/1
  Project_Module_outputs/6 -> [socParallelAssembly1]
  socParallelAssemblyMux/1 -> socParallelAssembly/1
  [socParallelAssembly1] -> socParallelAssemblyMux/1
  Project_Module_outputs/7 -> [vParallelAssembly1]
  vParallelAssemblyMux/1 -> vParallelAssembly/1
  [vParallelAssembly1] -> vParallelAssemblyMux/1
  connections:
  Project_Module/LConn2 -- +/RConn1
  Project_Module/RConn1 -- -/RConn1
  AmbH_To_1/LConn1 -- Project_Module/LConn1
  AmbH_From_1/LConn1 -- AmbH/RConn1

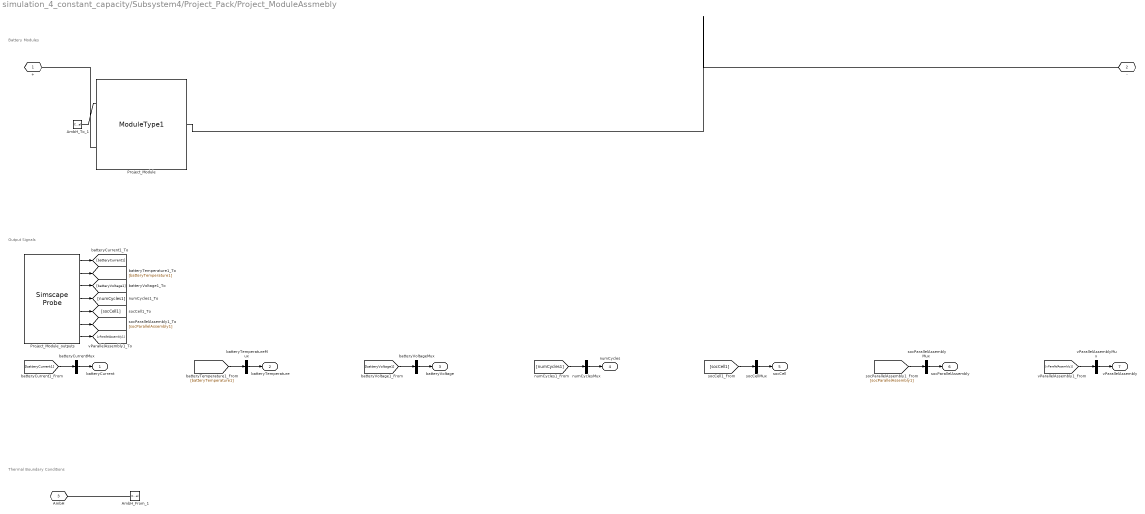
== system simulation_4_constant_capacity/Subsystem4/Project_Pack/Project_ModuleAssmebly ==
  note: Battery Modules
  note: Output Signals
  note: Thermal Boundary Conditions
  AmbH_From_1 : ConnectionLabel  Label=ambH_1
  AmbH_To_1 : ConnectionLabel  Label=ambH_1
  Project_Module : Batteries_lib/Modules/ModuleType1  BatteryCapacityCell=2.6 A*hr  ExtrapolationMethodCell=simscape.enum.extrapolation.nearest  SOCBreakpointsCell=[0 0.1 0.2 0.3 0.4 0.5 0.6 0.7 0.8 0.9 1]  TemperatureBreakpointsCell=[253.15 263.15 273.15 296.15 318.15] K  OpenCircuitVoltageThermalCell=|  VoltageRangeCell=[0, inf] V  ResistanceSOCBreakpointsCell=[0, .1, .25, .5, .75, .9, 1]  ResistanceTemperatureBreakpointsCell=[278, 293, 313] K  R0ThermalCell=[.0117, .0085, .009; .011, .0085, .009; .0114, .0087, .0092; .0107, .0082, .0088; .0107, .0083, .0091; .0113, .0085, .0089; .0116, .0085, .0089] Ohm  BatteryThermalMassCell=1840 J/K  AmbientResistance=25 K/W  socCell_specify=off  socCell_priority=High  socCell=0  socCell_nominal_specify=off  socCell_nominal_value=1  socCell_nominal_unit=1  batteryVoltage_specify=off  batteryVoltage_priority=None  batteryVoltage=0 V  batteryVoltage_nominal_specify=off  batteryVoltage_nominal_value=1  batteryVoltage_nominal_unit=V  batteryCurrent_specify=off  batteryCurrent_priority=None  batteryCurrent=0 A  batteryCurrent_nominal_specify=off  batteryCurrent_nominal_value=1  batteryCurrent_nominal_unit=A  numCycles_specify=off  numCycles_priority=High  numCycles=0  numCycles_nominal_specify=off  numCycles_nominal_value=1  numCycles_nominal_unit=1  batteryTemperature_specify=on  batteryTemperature_priority=High  batteryTemperature=283 K  batteryTemperature_nominal_specify=off  batteryTemperature_nominal_value=1  batteryTemperature_nominal_unit=K  vParallelAssembly_specify=off  vParallelAssembly_priority=None  vParallelAssembly=repmat(0, 10, 1) V  vParallelAssembly_nominal_specify=off  vParallelAssembly_nominal_value=1  vParallelAssembly_nominal_unit=V  socParallelAssembly_specify=off  socParallelAssembly_priority=None  socParallelAssembly=repmat(1, 10, 1)  socParallelAssembly_nominal_specify=off  socParallelAssembly_nominal_value=1  socParallelAssembly_nominal_unit=1
      | [3.00 3.00 3.00 3.00 3.00;
      |  3.07 3.23 3.40 3.65 3.70;
      |  3.09 3.31 3.49 3.67 3.71;
      |  3.10 3.38 3.54 3.70 3.73;
      |  3.11 3.44 3.59 3.72 3.75;
      |  3.13 3.50 3.65 3.75 3.78;
      |  3.15 3.55 3.70 3.80 3.83;
      |  3.19 3.61 3.76 3.87 3.90;
      |  3.24 3.69 3.82 3.95 3.98;
      |  3.34 3.78 3.90 4.02 4.03;
      |  3.59 3.97 4.10 4.16 4.16] V
  Project_Module_outputs : SimscapeProbe  BoundBlock=1241  Variables="{\"batteryCurrent\":{\"Probing\":\"ON\"},\"batteryTemperature\":{\"Probing\":\"ON\"},\"batteryVoltage\":{\"Probing\":\"ON\"},\"numCycles\":{\"Probing\":\"ON\"},\"socCell\":{\"Probing\":\"ON\"},\"socParallelAssembly\":{\"Probing\":\"ON\"},\"vParallelAssembly\":{\"Probing\":\"ON\"}}"
  batteryCurrentMux : Mux  Inputs=1
  batteryTemperatureMux : Mux  Inputs=1
  batteryVoltageMux : Mux  Inputs=1
  numCyclesMux : Mux  Inputs=1
  socCellMux : Mux  Inputs=1
  socParallelAssemblyMux : Mux  Inputs=1
  vParallelAssemblyMux : Mux  Inputs=1
  + : PMIOPort  Side=Left
  - : PMIOPort  Port=2  Side=Right
  AmbH : PMIOPort  Port=3  Side=Right  ConnectionType=Connection: foundation.thermal.thermal
  batteryCurrent : Outport
  batteryTemperature : Outport  Port=2
  batteryVoltage : Outport  Port=3
  numCycles : Outport  Port=4
  socCell : Outport  Port=5
  socParallelAssembly : Outport  Port=6
  vParallelAssembly : Outport  Port=7
  wires:
  Project_Module_outputs/1 -> [batteryCurrent1]
  batteryCurrentMux/1 -> batteryCurrent/1
  [batteryCurrent1] -> batteryCurrentMux/1
  Project_Module_outputs/2 -> [batteryTemperature1]
  batteryTemperatureMux/1 -> batteryTemperature/1
  [batteryTemperature1] -> batteryTemperatureMux/1
  Project_Module_outputs/3 -> [batteryVoltage1]
  batteryVoltageMux/1 -> batteryVoltage/1
  [batteryVoltage1] -> batteryVoltageMux/1
  Project_Module_outputs/4 -> [numCycles1]
  numCyclesMux/1 -> numCycles/1
  [numCycles1] -> numCyclesMux/1
  Project_Module_outputs/5 -> [socCell1]
  socCellMux/1 -> socCell/1
  [socCell1] -> socCellMux/1
  Project_Module_outputs/6 -> [socParallelAssembly1]
  socParallelAssemblyMux/1 -> socParallelAssembly/1
  [socParallelAssembly1] -> socParallelAssemblyMux/1
  Project_Module_outputs/7 -> [vParallelAssembly1]
  vParallelAssemblyMux/1 -> vParallelAssembly/1
  [vParallelAssembly1] -> vParallelAssemblyMux/1
  connections:
  Project_Module/LConn2 -- +/RConn1
  Project_Module/RConn1 -- -/RConn1
  AmbH_To_1/LConn1 -- Project_Module/LConn1
  AmbH_From_1/LConn1 -- AmbH/RConn1

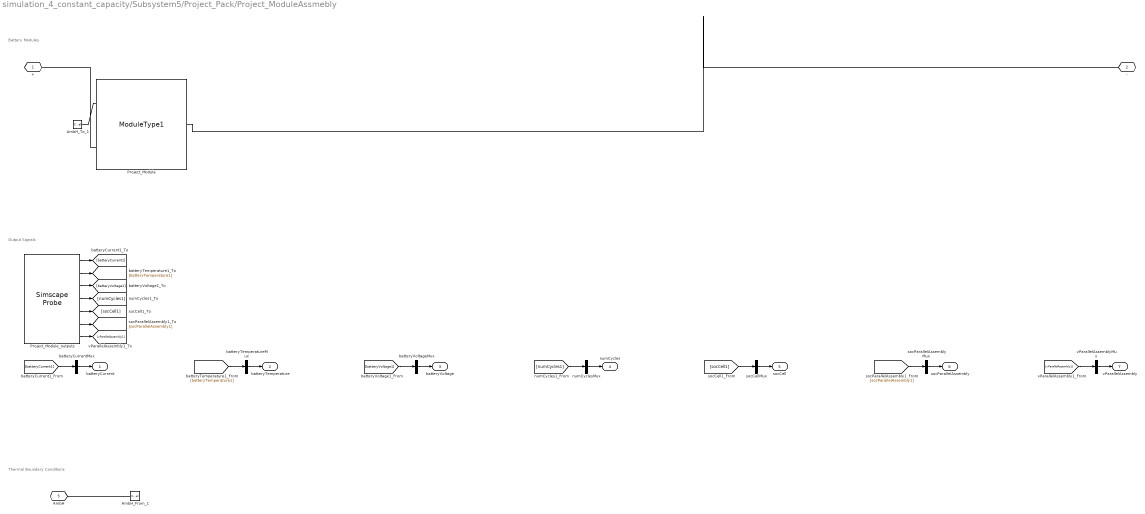
== system simulation_4_constant_capacity/Subsystem5/Project_Pack/Project_ModuleAssmebly ==
  note: Battery Modules
  note: Output Signals
  note: Thermal Boundary Conditions
  AmbH_From_1 : ConnectionLabel  Label=ambH_1
  AmbH_To_1 : ConnectionLabel  Label=ambH_1
  Project_Module : Batteries_lib/Modules/ModuleType1  BatteryCapacityCell=2.6 A*hr  ExtrapolationMethodCell=simscape.enum.extrapolation.nearest  SOCBreakpointsCell=[0 0.1 0.2 0.3 0.4 0.5 0.6 0.7 0.8 0.9 1]  TemperatureBreakpointsCell=[253.15 263.15 273.15 296.15 318.15] K  OpenCircuitVoltageThermalCell=|  VoltageRangeCell=[0, inf] V  ResistanceSOCBreakpointsCell=[0, .1, .25, .5, .75, .9, 1]  ResistanceTemperatureBreakpointsCell=[278, 293, 313] K  R0ThermalCell=[.0117, .0085, .009; .011, .0085, .009; .0114, .0087, .0092; .0107, .0082, .0088; .0107, .0083, .0091; .0113, .0085, .0089; .0116, .0085, .0089] Ohm  BatteryThermalMassCell=1840 J/K  AmbientResistance=25 K/W  socCell_specify=off  socCell_priority=High  socCell=0  socCell_nominal_specify=off  socCell_nominal_value=1  socCell_nominal_unit=1  batteryVoltage_specify=off  batteryVoltage_priority=None  batteryVoltage=0 V  batteryVoltage_nominal_specify=off  batteryVoltage_nominal_value=1  batteryVoltage_nominal_unit=V  batteryCurrent_specify=off  batteryCurrent_priority=None  batteryCurrent=0 A  batteryCurrent_nominal_specify=off  batteryCurrent_nominal_value=1  batteryCurrent_nominal_unit=A  numCycles_specify=off  numCycles_priority=High  numCycles=0  numCycles_nominal_specify=off  numCycles_nominal_value=1  numCycles_nominal_unit=1  batteryTemperature_specify=on  batteryTemperature_priority=High  batteryTemperature=333 K  batteryTemperature_nominal_specify=off  batteryTemperature_nominal_value=1  batteryTemperature_nominal_unit=K  vParallelAssembly_specify=off  vParallelAssembly_priority=None  vParallelAssembly=repmat(0, 10, 1) V  vParallelAssembly_nominal_specify=off  vParallelAssembly_nominal_value=1  vParallelAssembly_nominal_unit=V  socParallelAssembly_specify=off  socParallelAssembly_priority=None  socParallelAssembly=repmat(1, 10, 1)  socParallelAssembly_nominal_specify=off  socParallelAssembly_nominal_value=1  socParallelAssembly_nominal_unit=1
      | [3.00 3.00 3.00 3.00 3.00;
      |  3.07 3.23 3.40 3.65 3.70;
      |  3.09 3.31 3.49 3.67 3.71;
      |  3.10 3.38 3.54 3.70 3.73;
      |  3.11 3.44 3.59 3.72 3.75;
      |  3.13 3.50 3.65 3.75 3.78;
      |  3.15 3.55 3.70 3.80 3.83;
      |  3.19 3.61 3.76 3.87 3.90;
      |  3.24 3.69 3.82 3.95 3.98;
      |  3.34 3.78 3.90 4.02 4.03;
      |  3.59 3.97 4.10 4.16 4.16] V
  Project_Module_outputs : SimscapeProbe  BoundBlock=1357  Variables="{\"batteryCurrent\":{\"Probing\":\"ON\"},\"batteryTemperature\":{\"Probing\":\"ON\"},\"batteryVoltage\":{\"Probing\":\"ON\"},\"numCycles\":{\"Probing\":\"ON\"},\"socCell\":{\"Probing\":\"ON\"},\"socParallelAssembly\":{\"Probing\":\"ON\"},\"vParallelAssembly\":{\"Probing\":\"ON\"}}"
  batteryCurrentMux : Mux  Inputs=1
  batteryTemperatureMux : Mux  Inputs=1
  batteryVoltageMux : Mux  Inputs=1
  numCyclesMux : Mux  Inputs=1
  socCellMux : Mux  Inputs=1
  socParallelAssemblyMux : Mux  Inputs=1
  vParallelAssemblyMux : Mux  Inputs=1
  + : PMIOPort  Side=Left
  - : PMIOPort  Port=2  Side=Right
  AmbH : PMIOPort  Port=3  Side=Right  ConnectionType=Connection: foundation.thermal.thermal
  batteryCurrent : Outport
  batteryTemperature : Outport  Port=2
  batteryVoltage : Outport  Port=3
  numCycles : Outport  Port=4
  socCell : Outport  Port=5
  socParallelAssembly : Outport  Port=6
  vParallelAssembly : Outport  Port=7
  wires:
  Project_Module_outputs/1 -> [batteryCurrent1]
  batteryCurrentMux/1 -> batteryCurrent/1
  [batteryCurrent1] -> batteryCurrentMux/1
  Project_Module_outputs/2 -> [batteryTemperature1]
  batteryTemperatureMux/1 -> batteryTemperature/1
  [batteryTemperature1] -> batteryTemperatureMux/1
  Project_Module_outputs/3 -> [batteryVoltage1]
  batteryVoltageMux/1 -> batteryVoltage/1
  [batteryVoltage1] -> batteryVoltageMux/1
  Project_Module_outputs/4 -> [numCycles1]
  numCyclesMux/1 -> numCycles/1
  [numCycles1] -> numCyclesMux/1
  Project_Module_outputs/5 -> [socCell1]
  socCellMux/1 -> socCell/1
  [socCell1] -> socCellMux/1
  Project_Module_outputs/6 -> [socParallelAssembly1]
  socParallelAssemblyMux/1 -> socParallelAssembly/1
  [socParallelAssembly1] -> socParallelAssemblyMux/1
  Project_Module_outputs/7 -> [vParallelAssembly1]
  vParallelAssemblyMux/1 -> vParallelAssembly/1
  [vParallelAssembly1] -> vParallelAssemblyMux/1
  connections:
  Project_Module/LConn2 -- +/RConn1
  Project_Module/RConn1 -- -/RConn1
  AmbH_To_1/LConn1 -- Project_Module/LConn1
  AmbH_From_1/LConn1 -- AmbH/RConn1

== matlab function simulation_4_constant_capacity/Subsystem/Mean ==
  data: u input; y output
function y = fcn(u)

y = mean(u);

end

== matlab function simulation_4_constant_capacity/Subsystem/ODPC ==
  data: output_current output; charging_enabled input; SOC input; CC_CV_current input
function output_current = fcn(charging_enabled,SOC,CC_CV_current)


%% If battery is in discharge mode and the battery is fully drained, 
%% do not output current. Otherwise, output current should be the same as 
%% the CC-CV controller set. 
if not(charging_enabled) && SOC<= 0
    output_current = 0;
else
    output_current = CC_CV_current;
end

== matlab function simulation_4_constant_capacity/Subsystem1/Mean ==
  data: u input; y output
function y = fcn(u)

y = mean(u);

end

== matlab function simulation_4_constant_capacity/Subsystem1/ODPC ==
  data: output_current output; charging_enabled input; SOC input; CC_CV_current input
function output_current = fcn(charging_enabled,SOC,CC_CV_current)


%% If battery is in discharge mode and the battery is fully drained, 
%% do not output current. Otherwise, output current should be the same as 
%% the CC-CV controller set. 
if not(charging_enabled) && SOC<= 0
    output_current = 0;
else
    output_current = CC_CV_current;
end

== matlab function simulation_4_constant_capacity/Subsystem2/Mean ==
  data: u input; y output
function y = fcn(u)

y = mean(u);

end

== matlab function simulation_4_constant_capacity/Subsystem2/ODPC ==
  data: output_current output; charging_enabled input; SOC input; CC_CV_current input
function output_current = fcn(charging_enabled,SOC,CC_CV_current)


%% If battery is in discharge mode and the battery is fully drained, 
%% do not output current. Otherwise, output current should be the same as 
%% the CC-CV controller set. 
if not(charging_enabled) && SOC<= 0
    output_current = 0;
else
    output_current = CC_CV_current;
end

== matlab function simulation_4_constant_capacity/Subsystem3/Mean ==
  data: u input; y output
function y = fcn(u)

y = mean(u);

end

== matlab function simulation_4_constant_capacity/Subsystem3/ODPC ==
  data: output_current output; charging_enabled input; SOC input; CC_CV_current input
function output_current = fcn(charging_enabled,SOC,CC_CV_current)


%% If battery is in discharge mode and the battery is fully drained, 
%% do not output current. Otherwise, output current should be the same as 
%% the CC-CV controller set. 
if not(charging_enabled) && SOC<= 0
    output_current = 0;
else
    output_current = CC_CV_current;
end

== matlab function simulation_4_constant_capacity/Subsystem4/Mean ==
  data: u input; y output
function y = fcn(u)

y = mean(u);

end

== matlab function simulation_4_constant_capacity/Subsystem4/ODPC ==
  data: output_current output; charging_enabled input; SOC input; CC_CV_current input
function output_current = fcn(charging_enabled,SOC,CC_CV_current)


%% If battery is in discharge mode and the battery is fully drained, 
%% do not output current. Otherwise, output current should be the same as 
%% the CC-CV controller set. 
if not(charging_enabled) && SOC<= 0
    output_current = 0;
else
    output_current = CC_CV_current;
end

== matlab function simulation_4_constant_capacity/Subsystem5/Mean ==
  data: u input; y output
function y = fcn(u)

y = mean(u);

end

== matlab function simulation_4_constant_capacity/Subsystem5/ODPC ==
  data: output_current output; charging_enabled input; SOC input; CC_CV_current input
function output_current = fcn(charging_enabled,SOC,CC_CV_current)


%% If battery is in discharge mode and the battery is fully drained, 
%% do not output current. Otherwise, output current should be the same as 
%% the CC-CV controller set. 
if not(charging_enabled) && SOC<= 0
    output_current = 0;
else
    output_current = CC_CV_current;
end
